simulink model "GuidanceLaw"  (R2023b)
settings: Solver=ode4  StartTime=0.0  StopTime=400  FixedStep=0.05  RelTol=1e-3
values from neighbouring files (symbols this model uses):
  APCMD_TYPE : value not decoded    [apDataDictionary.sldd]
  missionRoutePlan_struct = struct(      'validWpNum_u8', uint8(5),      'missionRoute_struct', repmat(wpDefault_struct, double(maxWpNum_u8), 1))    [initMissionRoutePlan_MC.m]
  MSSN_TYPE : value not decoded    [apDataDictionary.sldd]
  setPoint_struct = struct('lat_deg_d',double(31.200000),'lon_deg_d',double(121.500000),'alt_m_f',single(100),'yaw_deg_f',single(0))    [APTest.m]
undefined symbols (not defined in the file or in its folder): apParams
libraries: simulink x13, simulink_extras x3
(part 3 of 7)

== system GuidanceLaw/Subsystem/wpMssnHandle/GuiLaw/mcSpdGuidance/vuCmdLimit ==
  vuCmd_mps_f : Inport
  perfParams_struct : Inport  Port=2  OutDataTypeStr=Bus: perfParamBus
  curVu_mps_f : Inport  Port=3
  reset_b : Inport  Port=4
  Add : Sum  Inputs=+-
  Add1 : Sum
  Bus Selector : BusSelector  OutputSignals=maxVz_mps_f,minVz_mps_f,maxAz_mps2_f,minAz_mps2_f
  Constant : Constant  Value=apParams.dt_s_f  OutDataTypeStr=single
  Constant1 : Constant  Value=apParams.dt_s_f  OutDataTypeStr=single
  Delay : Delay  DelayLength=1
  Product : Product
  Product1 : Product
  Saturation Dynamic : simulink/Discontinuities/Saturation Dynamic  OutMin=[]  OutMax=[]  OutDataTypeStr=Inherit: Same as second input  OutDataType=fixdt(1, 16)  OutScaling=2^-10  DoSatur=off
  Saturation Dynamic2 : simulink/Discontinuities/Saturation Dynamic  OutMin=[]  OutMax=[]  OutDataTypeStr=Inherit: Same as second input  OutDataType=fixdt(1, 16)  OutScaling=2^-10  DoSatur=off
  Switch : Switch  Criteria=u2 > Threshold  SaturateOnIntegerOverflow=off  InputSameDT=off
  vuCmdLimit_mps_f : Outport
  wires:
  [vuCmdPre_mps_f] -> Switch/3
  [reset_b] -> Switch/2
  [curVu_mps_f] -> Switch/1
  Add/1 -> Saturation Dynamic/2
  Constant/1 -> Product/1
  Product/1 -> Saturation Dynamic/1
  Product1/1 -> Saturation Dynamic/3
  Constant1/1 -> Product1/2
  perfParams_struct/1 -> Bus Selector/1
  Bus Selector/1 -> [maxVu_mps_f]  "<maxVz_mps_f>"
  Bus Selector/2 -> [minVu_mps_f]  "<minVz_mps_f>"
  Bus Selector/3 -> [maxAu_mps_f]  "<maxAz_mps2_f>"
  Bus Selector/4 -> [minAu_mps_f]  "<minAz_mps2_f>"
  [maxAu_mps_f] -> Product/2
  [minAu_mps_f] -> Product1/1
  Saturation Dynamic/1 -> Add1/1
  vuCmd_mps_f/1 -> [vuCmd_mps_f]  "vuCmd_mps_f"
  [vuCmd_mps_f] -> Add/1
  Add1/1 -> Saturation Dynamic2/2
  [maxVu_mps_f] -> Saturation Dynamic2/1
  [minVu_mps_f] -> Saturation Dynamic2/3
  Saturation Dynamic2/1 -> Delay/1, vuCmdLimit_mps_f/1
  Delay/1 -> [vuCmdPre_mps_f]
  curVu_mps_f/1 -> [curVu_mps_f]
  reset_b/1 -> [reset_b]  "reset_b"
  Switch/1 -> Add1/2, Add/2

== system GuidanceLaw/Subsystem/wpMssnHandle/GuiLaw/mcSpdGuidance/vxCmdLimit ==
  vxCmd_mps_f : Inport
  perfParams_struct : Inport  Port=2  OutDataTypeStr=Bus: perfParamBus
  curVx_mps_f : Inport  Port=3
  reset_b : Inport  Port=4
  Add : Sum  Inputs=+-
  Add1 : Sum
  Bus Selector : BusSelector  OutputSignals=maxVx_mps_f,minVx_mps_f,maxAx_mps2_f,minAx_mps2_f
  Constant : Constant  Value=apParams.dt_s_f  OutDataTypeStr=single
  Constant1 : Constant  Value=apParams.dt_s_f  OutDataTypeStr=single
  Delay : Delay  DelayLength=1
  Product : Product
  Product1 : Product
  Saturation Dynamic : simulink/Discontinuities/Saturation Dynamic  OutMin=[]  OutMax=[]  OutDataTypeStr=Inherit: Same as second input  OutDataType=fixdt(1, 16)  OutScaling=2^-10  DoSatur=off
  Saturation Dynamic2 : simulink/Discontinuities/Saturation Dynamic  OutMin=[]  OutMax=[]  OutDataTypeStr=Inherit: Same as second input  OutDataType=fixdt(1, 16)  OutScaling=2^-10  DoSatur=off
  Switch : Switch  Criteria=u2 > Threshold  SaturateOnIntegerOverflow=off  InputSameDT=off
  vxCmdLimit_mps_f : Outport
  wires:
  [vxCmdPre_mps_f] -> Switch/3
  [reset_b] -> Switch/2
  [curVx_mps_f] -> Switch/1
  Add/1 -> Saturation Dynamic/2
  Constant/1 -> Product/1
  Product/1 -> Saturation Dynamic/1
  Product1/1 -> Saturation Dynamic/3
  Constant1/1 -> Product1/2
  perfParams_struct/1 -> Bus Selector/1
  Bus Selector/1 -> [maxVx_mps_f]  "<maxVx_mps_f>"
  Bus Selector/2 -> [minVx_mps_f]  "<minVx_mps_f>"
  Bus Selector/3 -> [maxAx_mps_f]  "<maxAx_mps2_f>"
  Bus Selector/4 -> [minAx_mps_f]  "<minAx_mps2_f>"
  [maxAx_mps_f] -> Product/2
  [minAx_mps_f] -> Product1/1
  Saturation Dynamic/1 -> Add1/1
  vxCmd_mps_f/1 -> [vxCmd_mps_f]
  [vxCmd_mps_f] -> Add/1
  Add1/1 -> Saturation Dynamic2/2
  [maxVx_mps_f] -> Saturation Dynamic2/1
  [minVx_mps_f] -> Saturation Dynamic2/3
  Saturation Dynamic2/1 -> Delay/1, vxCmdLimit_mps_f/1
  Delay/1 -> [vxCmdPre_mps_f]
  curVx_mps_f/1 -> [curVx_mps_f]
  reset_b/1 -> [reset_b]
  Switch/1 -> Add1/2, Add/2

== system GuidanceLaw/Subsystem/wpMssnHandle/GuiLaw/mcSpdGuidance/vyCmdLimit ==
  vyCmd_mps_f : Inport
  perfParams_struct : Inport  Port=2  OutDataTypeStr=Bus: perfParamBus
  curVy_mps_f : Inport  Port=3
  reset_b : Inport  Port=4
  Add : Sum  Inputs=+-
  Add1 : Sum
  Bus Selector : BusSelector  OutputSignals=maxVy_mps_f,minVy_mps_f,maxAy_mps2_f,minAy_mps2_f
  Constant : Constant  Value=apParams.dt_s_f  OutDataTypeStr=single
  Constant1 : Constant  Value=apParams.dt_s_f  OutDataTypeStr=single
  Delay : Delay  DelayLength=1
  Product : Product
  Product1 : Product
  Saturation Dynamic : simulink/Discontinuities/Saturation Dynamic  OutMin=[]  OutMax=[]  OutDataTypeStr=Inherit: Same as second input  OutDataType=fixdt(1, 16)  OutScaling=2^-10  DoSatur=off
  Saturation Dynamic2 : simulink/Discontinuities/Saturation Dynamic  OutMin=[]  OutMax=[]  OutDataTypeStr=Inherit: Same as second input  OutDataType=fixdt(1, 16)  OutScaling=2^-10  DoSatur=off
  Switch : Switch  Criteria=u2 > Threshold  SaturateOnIntegerOverflow=off  InputSameDT=off
  vyCmdLimit_mps_f : Outport
  wires:
  [vyCmdPre_mps_f] -> Switch/3
  [reset_b] -> Switch/2
  [curVy_mps_f] -> Switch/1
  Add/1 -> Saturation Dynamic/2
  Constant/1 -> Product/1
  Product/1 -> Saturation Dynamic/1
  Product1/1 -> Saturation Dynamic/3
  Constant1/1 -> Product1/2
  perfParams_struct/1 -> Bus Selector/1
  Bus Selector/1 -> [maxVy_mps_f]  "<maxVy_mps_f>"
  Bus Selector/2 -> [minVy_mps_f]  "<minVy_mps_f>"
  Bus Selector/3 -> [maxAy_mps_f]  "<maxAy_mps2_f>"
  Bus Selector/4 -> [minAy_mps_f]  "<minAy_mps2_f>"
  [maxAy_mps_f] -> Product/2
  [minAy_mps_f] -> Product1/1
  Saturation Dynamic/1 -> Add1/1
  vyCmd_mps_f/1 -> [vyCmd_mps_f]
  [vyCmd_mps_f] -> Add/1
  Add1/1 -> Saturation Dynamic2/2
  [maxVy_mps_f] -> Saturation Dynamic2/1
  [minVy_mps_f] -> Saturation Dynamic2/3
  Saturation Dynamic2/1 -> Delay/1, vyCmdLimit_mps_f/1
  Delay/1 -> [vyCmdPre_mps_f]
  curVy_mps_f/1 -> [curVy_mps_f]
  reset_b/1 -> [reset_b]
  Switch/1 -> Add/2, Add1/2

== system GuidanceLaw/Subsystem/wpMssnHandle/GuiLaw/yawGuidance/yawCmdLimit ==
  yawCmd_deg_f : Inport
  perfParams_struct : Inport  Port=2  OutDataTypeStr=Bus: perfParamBus
  curYaw_deg_f : Inport  Port=3
  reset_b : Inport  Port=4
  Add : Sum  Inputs=+-
  Add1 : Sum
  Bus Selector : BusSelector  OutputSignals=maxYawAngleRate_dps_f,minYawAngleRate_dps_f
  Constant : Constant  Value=apParams.dt_s_f  OutDataTypeStr=single
  Constant1 : Constant  Value=apParams.dt_s_f  OutDataTypeStr=single
  Delay : Delay  DelayLength=1
  Product : Product
  Product1 : Product
  Saturation Dynamic : simulink/Discontinuities/Saturation Dynamic  OutMin=[]  OutMax=[]  OutDataTypeStr=Inherit: Same as second input  OutDataType=fixdt(1, 16)  OutScaling=2^-10  DoSatur=off
  Switch : Switch  Criteria=u2 > Threshold  SaturateOnIntegerOverflow=off  InputSameDT=off
  cldWrap180 : MATLAB Function  TreatAsAtomicUnit=on
  cldWrap1801 : MATLAB Function  TreatAsAtomicUnit=on
  yawCmdLimit_deg_f : Outport
  wires:
  [yawCmdPre_mps_f] -> Switch/3
  [reset_b] -> Switch/2
  [curYaw_deg_f] -> Switch/1
  Constant/1 -> Product/1
  Product/1 -> Saturation Dynamic/1
  Product1/1 -> Saturation Dynamic/3
  Constant1/1 -> Product1/2
  perfParams_struct/1 -> Bus Selector/1
  Bus Selector/1 -> [maxYawRate_dps_f]  "<maxYawAngleRate_dps_f>"
  Bus Selector/2 -> [minYawRate_dps_f]  "<minYawAngleRate_dps_f>"
  [maxYawRate_dps_f] -> Product/2
  [minYawRate_dps_f] -> Product1/1
  Saturation Dynamic/1 -> Add1/1
  yawCmd_deg_f/1 -> [yawCmd_deg_f]
  [yawCmd_deg_f] -> Add/1
  cldWrap1801/1(y) -> Delay/1, yawCmdLimit_deg_f/1
  Delay/1 -> [yawCmdPre_mps_f]
  curYaw_deg_f/1 -> [curYaw_deg_f]
  reset_b/1 -> [reset_b]
  Switch/1 -> Add1/2, Add/2
  cldWrap180/1(y) -> Saturation Dynamic/2
  Add/1 -> cldWrap180/1(u)
  Add1/1 -> cldWrap1801/1(u)

== system GuidanceLaw/Subsystem/wpMssnHandle/WaypointArrivalState/hoverYawJudge/YawAlignJudge ==
  note: 仅当 isHoverPosReach_b=true 时执行。
      | 禁用时输出复位为 false，重新使能时内部状态复位。
  curPosNEU_m_f : Inport
  curYaw_deg_f : Inport  Port=2
  reset_b : Inport  Port=3
  nextWp_struct : Inport  Port=4
  curWp_struct : Inport  Port=5
  Enable : EnablePort  StatesWhenEnabling=reset
  Bus Selector : BusSelector  OutputSignals=yawType_u8,yaw_deg_f,posN_m_f,posE_m_f
  Bus Selector1 : BusSelector  OutputSignals=posN_m_f,posE_m_f
  Constant1 : Constant  Value=apParams.hoverYawJudge.holdTimeCond_s_f  OutDataTypeStr=single
  Constant2 : Constant  Value=apParams.hoverYawJudge.minYawDirDist_m_f  OutDataTypeStr=single
  Constant21 : Constant  Value=apParams.dt_s_f  OutDataTypeStr=single
  Constant9 : Constant  Value=apParams.hoverYawJudge.yawTolerance_deg_f  OutDataTypeStr=single
  Selector : Selector  InputPortWidth=3  IndexOptions=Index vector (dialog)  Indices=[1 2]  OutputSizes=1
  Terminator : Terminator
  Vector Concatenate : Concatenate
  Vector Concatenate1 : Concatenate
  YawJudgeAlgorithmBlock : MATLAB Function  TreatAsAtomicUnit=on
  hoverYawJudge_b : Outport  OutDataTypeStr=boolean  OutputWhenDisabled=reset  InitialOutput=false
  wires:
  YawJudgeAlgorithmBlock/1(hoverYawJudge_b) -> hoverYawJudge_b/1
  YawJudgeAlgorithmBlock/2(yawCmd_deg_f) -> Terminator/1
  curYaw_deg_f/1 -> YawJudgeAlgorithmBlock/3(curYaw_deg_f)
  Constant21/1 -> YawJudgeAlgorithmBlock/7(dt_s_f)
  Constant9/1 -> YawJudgeAlgorithmBlock/8(yawErrAccept_deg_f)
  Constant1/1 -> YawJudgeAlgorithmBlock/9(holdTimeYaw_s_f)
  Constant2/1 -> YawJudgeAlgorithmBlock/10(minYawDirDist_m_f)
  reset_b/1 -> YawJudgeAlgorithmBlock/6(reset_b)
  nextWp_struct/1 -> Bus Selector/1
  Bus Selector/1 -> [nextWpYawType_u8]  "<yawType_u8>"
  [nextWpYawType_u8] -> YawJudgeAlgorithmBlock/4(nextWpYawType_u8)
  Bus Selector/2 -> [nextWpYaw_deg_f]  "<yaw_deg_f>"
  [nextWpYaw_deg_f] -> YawJudgeAlgorithmBlock/5(nextWpYaw_deg_f)
  Bus Selector/3 -> Vector Concatenate/1  "<posN_m_f>"
  Bus Selector/4 -> Vector Concatenate/2  "<posE_m_f>"
  Vector Concatenate/1 -> [nextWpNE_m_f]
  [nextWpNE_m_f] -> YawJudgeAlgorithmBlock/2(nextWpNE_m_f)
  curWp_struct/1 -> Bus Selector1/1
  Bus Selector1/1 -> Vector Concatenate1/1  "<posN_m_f>"
  Bus Selector1/2 -> Vector Concatenate1/2  "<posE_m_f>"
  Vector Concatenate1/1 -> [curWpNE_m_f]
  [curWpNE_m_f] -> YawJudgeAlgorithmBlock/11(curWpNE_m_f)
  curPosNEU_m_f/1 -> [curPosNEU_m_f]
  Selector/1 -> YawJudgeAlgorithmBlock/1(curPosNE_m_f)
  [curPosNEU_m_f] -> Selector/1

== matlab function GuidanceLaw/Subsystem/wpMssnHandle/GuiLaw/L1CirleGuidance/L1CirleGuidance ==
  data: kdCir_f input; rollCmd_deg_f output; ktCir_f input; curVelNE_mps_f input; curPosNE_mps_f input; velXY_min input; G_mps2_f input; curPitch_deg_f input; curGpPosN_m_f input; curWpPosE_m_f input; curWpRadius_m_f input; circle_radius_min input; curYaw_deg_f input
function rollCmd_deg_f = l1CircleGuidance(kdCir_f, ktCir_f, curVelNE_mps_f, curPosNE_mps_f, velXY_min, G_mps2_f, curPitch_deg_f, curGpPosN_m_f, ...
    curWpPosE_m_f, curWpRadius_m_f, circle_radius_min, curYaw_deg_f)
%L1圆弧导引算法
%
% 优化内容：
% 1. 全部内部计算统一为single，便于Simulink代码生成。
% 2. 增加周期、阻尼、重力、半径、速度和距离的有效性保护。
% 3. 避免飞机位于圆心时出现除零。
% 4. 使用显式二维运算替代norm/dot/辅助函数，计算量和类型更可控。
% 5. 低速时使用当前偏航方向构造等效速度。
% 6. 启用30 deg滚转角限幅，可按机型修改ROLL_LIMIT_DEG。
% 7. 圆周向心加速度使用真实有效半径，不再隐式限制为至少1 m。
%
% 输入：
%   curVelNE_mps_f = [v_N, v_E]，m/s，1×2
%   curPosNE_mps_f = [p_N, p_E]，m，1×2
%   curWpRadius_m_f > 0：顺时针；< 0：逆时针
%
%#codegen

%--------------------------- 常量定义 ------------------------------------
ZERO = single(0);
ONE  = single(1);
TWO  = single(2);
FOUR = single(4);

PI_S      = single(pi);
DEG2RAD_S = PI_S / single(180);
RAD2DEG_S = single(180) / PI_S;

EPS_PARAM = single(1.0e-6);
EPS_DIST  = single(1.0e-3);

% 默认安全输出
rollCmd_deg_f = ZERO;

%--------------------------- 输入类型统一 --------------------------------
Kd       = single(kdCir_f);
T_period = single(ktCir_f);
g        = single(G_mps2_f);

vN = single(curVelNE_mps_f(1));
vE = single(curVelNE_mps_f(2));

posN = single(curPosNE_mps_f(1));
posE = single(curPosNE_mps_f(2));

centerN = single(curGpPosN_m_f);
centerE = single(curWpPosE_m_f);

radius_cmd = single(curWpRadius_m_f);
radius_min = abs(single(circle_radius_min));
v_min      = max(single(velXY_min), ZERO);

yaw_rad   = single(curYaw_deg_f)   * DEG2RAD_S;
pitch_rad = single(curPitch_deg_f) * DEG2RAD_S;

%--------------------------- 参数有效性检查 ------------------------------
if Kd <= EPS_PARAM || T_period <= EPS_PARAM || g <= EPS_PARAM
    return;
end

% 带符号半径决定盘旋方向
if radius_cmd > EPS_PARAM
    loiter_direction = ONE;       % 顺时针
elseif radius_cmd < -EPS_PARAM
    loiter_direction = -ONE;      % 逆时针
else
    % 半径无方向信息，禁止产生不确定的盘旋指令
    return;
end

radius = max(abs(radius_cmd), max(radius_min, EPS_DIST));

%--------------------------- 地速处理 ------------------------------------
groundspeed_sq = vN * vN + vE * vE;
groundspeed = sqrt(max(groundspeed_sq, ZERO));

% 低速时，用当前偏航方向构造最小等效地速
if groundspeed < v_min
    groundspeed = v_min;
    vN = groundspeed * cos(yaw_rad);
    vE = groundspeed * sin(yaw_rad);
end

% 速度仍接近0时无法形成有效L1导引
if groundspeed <= EPS_PARAM
    return;
end

%--------------------------- L1参数计算 ----------------------------------
omega = TWO * PI_S / T_period;
K_c   = omega * omega;
K_v   = TWO * Kd * omega;
k_r   = Kd * T_period / PI_S;
K_L1  = FOUR * Kd * Kd;

L1 = k_r * groundspeed;
if L1 <= EPS_PARAM
    return;
end

%--------------------------- 圆心方向计算 --------------------------------
% 位置指向圆心：P -> C
dN = centerN - posN;
dE = centerE - posE;

distance_sq = dN * dN + dE * dE;
distance_to_center = sqrt(max(distance_sq, ZERO));

if distance_to_center > EPS_DIST
    inv_distance = ONE / distance_to_center;
    unitN = dN * inv_distance;
    unitE = dE * inv_distance;
else
    % 飞机恰好位于圆心，P->C方向不确定。
    % 构造一个与当前速度垂直、且与目标旋转方向一致的单位方向，
    % 使算法能够主动建立盘旋，而不是产生NaN。
    inv_speed = ONE / groundspeed;
    unitN = -loiter_direction * vE * inv_speed;
    unitE =  loiter_direction * vN * inv_speed;
    distance_to_center = ZERO;
end

% 速度在P->C方向上的横向和纵向分量
xtrackVelCap = vN * unitE - vE * unitN;
ltrackVelCap = vN * unitN + vE * unitE;

%--------------------------- 圆心捕获L1导引 ------------------------------
eta = atan2(xtrackVelCap, ltrackVelCap);
eta = min(max(eta, -PI_S / TWO), PI_S / TWO);

latAccDemLine = K_L1 * groundspeed * groundspeed / L1 * sin(eta);

%--------------------------- 圆航线跟踪 ----------------------------------
% 径向误差：圆外为正，圆内为负
xtrackErrCirc = distance_to_center - radius;

% 径向速度：向圆外运动为正，向圆心运动为负
xtrackVelCirc = -ltrackVelCap;

% 径向PD修正项
latAccDemCircPD = K_c * xtrackErrCirc + K_v * xtrackVelCirc;

% 与目标盘旋方向一致的切向速度
velTangent = loiter_direction * xtrackVelCap;

% 当前速度方向与目标盘旋方向相反时，
% 禁止PD项继续诱导飞机向反方向旋转
if ltrackVelCap < ZERO && velTangent < ZERO
    latAccDemCircPD = max(ZERO, latAccDemCircPD);
end

% 圆周跟踪指令 = 径向PD修正 + 向心加速度前馈
latAccDemCirc = loiter_direction * (latAccDemCircPD + velTangent * velTangent / radius);

%--------------------------- 捕获/跟踪切换 -------------------------------
% 飞机位于圆外时，若圆心捕获指令更温和，则采用捕获指令；
% 否则直接采用圆航线跟踪指令。
if xtrackErrCirc > ZERO && loiter_direction * latAccDemLine < loiter_direction * latAccDemCirc
    lateral_accel = latAccDemLine;
else
    lateral_accel = latAccDemCirc;
end

%--------------------------- 滚转角反算 ----------------------------------
roll_rad = atan(cos(pitch_rad) * lateral_accel / g);
rollCmd_deg_f = single(roll_rad * RAD2DEG_S);

end

== matlab function GuidanceLaw/Subsystem/wpMssnHandle/GuiLaw/L1LineGuidance/L1LineGuidance ==
  data: kdLine_f input; rollCmd_deg_f output; ktLine_f input; curVelNE_mps_f input; curPosNE_m_f input; velXY_min input; G_mps2_f input; curPitch_deg_f input; curGpPosN_m_f input; curGpPosE_m_f input; preGpPosN_m_f input; preGpPosE_m_f input; mssnType_u8 input; curYaw_deg_f input
function rollCmd_deg_f = l1LineGuidance(kdLine_f, ktLine_f, curVelNE_mps_f, curPosNE_m_f, velXY_min, G_mps2_f, curPitch_deg_f, curGpPosN_m_f, curGpPosE_m_f, preGpPosN_m_f, ...
    preGpPosE_m_f, mssnType_u8, curYaw_deg_f)
%#codegen
%
% 坐标约定：
%   水平面N-E坐标
%   curVelNE_mps_f = [VN, VE]
%   curPosNE_m_f   = [PN, PE]
%
% 输出：
%   rollCmd_deg_f，单位deg

%% 常量
PI_F       = single(3.14159265358979323846);
DEG2RAD_F  = single(0.01745329251994329577);
RAD2DEG_F  = single(57.2957795130823208768);

EPS_DIST   = single(1.0e-6);
EPS_SPEED  = single(1.0e-3);
EPS_G      = single(1.0e-3);

L1_MIN     = single(0.1);
SIN_45     = single(0.7071067811865476);
ETA_MAX    = single(0.5) * PI_F;
ANGLE_100  = single(100.0) * DEG2RAD_F;

rollCmd_deg_f = single(0.0);

%% 参数有效性保护
if (kdLine_f <= single(0.0)) || (ktLine_f <= single(0.0)) || (G_mps2_f <= EPS_G)
    return;
end

%% 读取当前位置、速度和航点
vN = curVelNE_mps_f(1);
vE = curVelNE_mps_f(2);

pN = curPosNE_m_f(1);
pE = curPosNE_m_f(2);

% 航段起点A
aN = preGpPosN_m_f;
aE = preGpPosE_m_f;

% 航段终点B
bN = curGpPosN_m_f;
bE = curGpPosE_m_f;

%% 计算当前地速
groundSpeedSq = vN * vN + vE * vE;
groundSpeed   = sqrt(groundSpeedSq);

% 最小地速限制
speedFloor = max(velXY_min, EPS_SPEED);

if groundSpeed < speedFloor
    groundSpeed = speedFloor;

    % 当前速度过小时，使用当前偏航角构造虚拟速度
    yaw_rad = curYaw_deg_f * DEG2RAD_F;

    vN = groundSpeed * cos(yaw_rad);
    vE = groundSpeed * sin(yaw_rad);
end

%% L1参数
k_r  = kdLine_f * ktLine_f / PI_F;
k_L1 = single(4.0) * kdLine_f * kdLine_f;

% L1距离增加下限保护
L1 = max(k_r * groundSpeed, L1_MIN);

%% 计算航段方向A->B
abN = bN - aN;
abE = bE - aE;

abLength = sqrt(abN * abN + abE * abE);

% 如果航段A、B重合，则退化为当前位置直接指向B
if abLength < EPS_DIST
    abN = bN - pN;
    abE = bE - pE;

    abLength = sqrt(abN * abN + abE * abE);

    % 当前位置也在B点，直接输出零
    if abLength < EPS_DIST
        return;
    end
end

% 航段方向单位向量
dirAbN = abN / abLength;
dirAbE = abE / abLength;

%% P指向A
paN = aN - pN;
paE = aE - pE;

distancePtoA = sqrt(paN * paN + paE * paE);

% A指向P
apN = -paN;
apE = -paE;

% 当前点在航段方向上的投影
trackDist = apN * dirAbN + apE * dirAbE;

%% P指向B
pbN = bN - pN;
pbE = bE - pE;

distancePtoB = sqrt(pbN * pbN + pbE * pbE);

%% 前倾飞行状态判断
% 如果项目中没有MSSN_TYPE枚举，需要将右侧替换为实际枚举值。
isForwardTilt = (mssnType_u8 == MSSN_TYPE.AUTO_FORWARD_TILT);

%% 判断是否位于A点后方
beforeARatio = trackDist / max(distancePtoA, single(1.0));

useDirectToA = (~isForwardTilt) && (distancePtoA > L1) && (beforeARatio < -SIN_45);

%% 判断是否位于B点外侧区域
useDirectToB = false;

if distancePtoB > EPS_DIST
    % B指向P的单位向量
    bpN = -pbN / distancePtoB;
    bpE = -pbE / distancePtoB;

    % BP到AB的有符号夹角
    crossBpAb = cross2(bpN, bpE, dirAbN, dirAbE);
    dotBpAb   = bpN * dirAbN + bpE * dirAbE;

    bpToAbBearing = atan2(crossBpAb, dotBpAb);

    useDirectToB = (~isForwardTilt) && (abs(bpToAbBearing) < ANGLE_100);
end

%% 计算导引角eta
if useDirectToA
    % 飞向A点
    targetN = paN / distancePtoA;
    targetE = paE / distancePtoA;

    eta = signedAngle(vN, vE, targetN, targetE);

elseif useDirectToB
    % 飞向B点
    targetN = pbN / distancePtoB;
    targetE = pbE / distancePtoB;

    eta = signedAngle(vN, vE, targetN, targetE);

else
    % 当前速度方向与航段方向的夹角
    eta2 = signedAngle(vN, vE, dirAbN, dirAbE);

    % 有符号横向航迹误差
    %
    % error_d = cross(A->P, A->B单位向量)
    error_d = cross2(apN, apE, dirAbN, dirAbE);

    % 横向误差转化为捕获角
    sineEta1 = error_d / L1;

    % 捕获角限制为±45°
    sineEta1 = constrain_scalar(sineEta1, -SIN_45, SIN_45);

    eta1 = asin(sineEta1);

    eta = eta1 + eta2;
end

%% 限制总导引角
eta = constrain_scalar(eta, -ETA_MAX, ETA_MAX);

%% 计算侧向加速度
lateralAccel = k_L1 * groundSpeed * groundSpeed / L1 * sin(eta);

%% 侧向加速度转换为滚转角
pitch_rad = curPitch_deg_f * DEG2RAD_F;

roll_rad = atan2(cos(pitch_rad) * lateralAccel, G_mps2_f);

rollCmd_deg_f = single(roll_rad * RAD2DEG_F);

end


function c = cross2(aN, aE, bN, bE)
% 二维叉乘
c = aN * bE - aE * bN;
end


function angle = signedAngle(aN, aE, bN, bE)
% 从向量a旋转到向量b的有符号夹角
crossValue = aN * bE - aE * bN;
dotValue   = aN * bN + aE * bE;

angle = atan2(crossValue, dotValue);
end


% function y = clampLimit(x, lowerLimit, upperLimit)
% % 上下限约束
% y = min(max(x, lowerLimit), upperLimit);
% end

== matlab function GuidanceLaw/Subsystem/wpMssnHandle/GuiLaw/mcSpdGuidance/mcTrajectoryGeneratorNEU/TrajectoryGeneratorNEU ==
  data: trajPosNEU_m_f output; curPosNEU_m_f input; curVelNEU_mps_f input; curAccNEU_mps2_f input; preWpNEU_m_f input; curWpNEU_m_f input; nextWpNEU_m_f input; velSpNEU_mps_f input; posVelValid_vec input; isHoverWp_b input; forceStop_b input; segSwitch_b input; newOriOldNEU_m_f input; dt_s_f input; reset_b input; paramNE_f input; trajVelNEU_mps_f output; trajAccNEU_mps2_f output; trajJerkNEU_mps3_f output; paramU_f input
function [trajPosNEU_m_f, trajVelNEU_mps_f, trajAccNEU_mps2_f, trajJerkNEU_mps3_f] = trajGeneratorNEU(curPosNEU_m_f, curVelNEU_mps_f, curAccNEU_mps2_f, preWpNEU_m_f, curWpNEU_m_f, nextWpNEU_m_f, ...
    velSpNEU_mps_f, posVelValid_vec, isHoverWp_b, forceStop_b, segSwitch_b, newOriOldNEU_m_f, dt_s_f, reset_b, paramNE_f, paramU_f)
%#codegen
%
% 功能：
% 生成NEU三轴jerk受限平滑轨迹，并进行N/E/U三轴S曲线时间同步。
%
% velSpNEU_mps_f：
% 1. 对应位置无效时，为纯速度目标；
% 2. 对应位置有效时，为位置导引速度上的速度前馈。
%
% posVelValid_vec：[posNEValid; velNEValid; posUValid; velUValid]
%
% paramNE_f：
% 1 最大水平jerk，[m/s^3]
% 2 最大水平加速度，[m/s^2]
% 3 最大水平速度，[m/s]
% 4 水平巡航速度，[m/s]
% 5 最大允许水平轨迹误差，[m]
% 6 水平航点接受半径，[m]
% 7 最小前视距离，[m]
% 8 转弯判断最小轨迹速度，[m/s]
% 9 转弯判断方向余弦阈值
% 10 前倾转换阶段旋翼水平速度，[m/s]
% 11 旋翼直线最小提前判定距离，[m]
% 12 旋翼直线最大提前判定距离，[m]
% 13 旋翼直线相邻航段长度限制比例，建议<=0.49
%
% paramU_f：
% 1 最大垂向jerk，[m/s^3]
% 2 爬升轨迹使用的最大垂向加速度幅值，[m/s^2]
% 3 下降轨迹使用的最大垂向加速度幅值，[m/s^2]
% 4 最大爬升速度，[m/s]
% 5 最大下降速度幅值，[m/s]
% 6 最大允许垂向轨迹误差，[m]
% 7 垂向航点接受半径，[m]
%
% 垂向非对称约束：
% 1. 根据未平滑垂向速度目标rawVelSpNEU_mps_f(3)的方向，选择一整套
%    垂向速度和加速度幅值约束；
% 2. 选定后，单轴S曲线规划器内部仍使用对称的+/-maxAcceleration约束；
% 3. rawVelSpU为0时保持上一套约束，避免停车附近反复切换。

%% 常量

smallValue_f = single(1.0e-6);
floatEpsilon_f = single(1.1920929e-7);
clampAccuracy_mps_f = single(0.5);

%% 最小持久状态
% 轨迹生成器每个周期都会根据当前状态重新规划S曲线，并在同一周期推进dt。
persistent trajAccStateNEU_mps2_f trajVelStateNEU_mps_f trajPosStateNEU_m_f
persistent selectedUConstraintModeState_i8
persistent preMaxSpeedNEState_mps_f
persistent turnJudgeDistState_m_f turnPassSpeedState_mps_f
persistent initialized_b

if isempty(initialized_b)
    initialized_b = false;

    trajAccStateNEU_mps2_f = single(zeros(3,1));
    trajVelStateNEU_mps_f = single(zeros(3,1));
    trajPosStateNEU_m_f = single(zeros(3,1));
    selectedUConstraintModeState_i8 = int8(0);
    preMaxSpeedNEState_mps_f = single(0.0);
    turnJudgeDistState_m_f = single(0.0);
    turnPassSpeedState_mps_f = single(0.0);
end

%% 参数读取
maxJerkNE_mps3_f = max(paramNE_f(1), smallValue_f);
maxAccNE_mps2_f = max(paramNE_f(2), smallValue_f);
maxVelNE_mps_f = max(paramNE_f(3), smallValue_f);
maxRouteSpeedNE_mps_f = constrain_scalar(paramNE_f(4), single(0.0), maxVelNE_mps_f);
maxTrajErrorNE_m_f = max(paramNE_f(5), smallValue_f);
horizonAptRadius_m_f = max(paramNE_f(6), smallValue_f);
minLookaheadDist_m_f = max(paramNE_f(7), horizonAptRadius_m_f);
turnMinSpeed_mps_f = max(paramNE_f(8), single(0.0));
turnCosThreshold_f = constrain_scalar(paramNE_f(9), single(-1.0), single(1.0));
fwdFixedSpd_mps_f = max(paramNE_f(10), smallValue_f);
minJudgeDistNE_m_f = max(paramNE_f(11), single(0.0));
maxJudgeDistNE_m_f = max(paramNE_f(12), minJudgeDistNE_m_f);
segmentLimitRatioNE_f = min(max(paramNE_f(13), single(0.0)), single(0.49));

maxJerkU_mps3_f = max(paramU_f(1), smallValue_f);
maxAccUp_mps2_f = max(paramU_f(2), smallValue_f);
maxAccDown_mps2_f = max(paramU_f(3), smallValue_f);
maxVelUp_mps_f = max(paramU_f(4), smallValue_f);
maxVelDown_mps_f = max(paramU_f(5), smallValue_f);
maxTrajErrorU_m_f = max(paramU_f(6), smallValue_f);
verticalAcceptanceRadius_m_f = max(paramU_f(7), smallValue_f);

axisMaxJerkNEU_mps3_f = single([maxJerkNE_mps3_f; maxJerkNE_mps3_f; maxJerkU_mps3_f]);

dtEff_s_f = max(dt_s_f, single(0.0));

%% 输入有效性
posNEValid_b = logical(posVelValid_vec(1));
velNEValid_b = logical(posVelValid_vec(2));
posUValid_b = logical(posVelValid_vec(3));
velUValid_b = logical(posVelValid_vec(4));

%% 初始化、复位或航段坐标系切换
if reset_b || ~initialized_b
    trajAccStateNEU_mps2_f = curAccNEU_mps2_f;
    trajVelStateNEU_mps_f = curVelNEU_mps_f;
    trajPosStateNEU_m_f = curPosNEU_m_f;

    trajAccStateNEU_mps2_f(1) = constrain_scalar(curAccNEU_mps2_f(1), -maxAccNE_mps2_f, maxAccNE_mps2_f);
    trajAccStateNEU_mps2_f(2) = constrain_scalar(curAccNEU_mps2_f(2), -maxAccNE_mps2_f, maxAccNE_mps2_f);
    trajAccStateNEU_mps2_f(3) = constrain_scalar(curAccNEU_mps2_f(3), -maxAccDown_mps2_f, maxAccUp_mps2_f);

    trajVelStateNEU_mps_f(1) = constrain_scalar(curVelNEU_mps_f(1), -maxVelNE_mps_f, maxVelNE_mps_f);
    trajVelStateNEU_mps_f(2) = constrain_scalar(curVelNEU_mps_f(2), -maxVelNE_mps_f, maxVelNE_mps_f);
    trajVelStateNEU_mps_f(3) = constrain_scalar(curVelNEU_mps_f(3), -maxVelDown_mps_f, maxVelUp_mps_f);

    % 1表示爬升约束，-1表示下降约束，0表示尚未选择方向并采用保守值。
    if curVelNEU_mps_f(3) > smallValue_f
        selectedUConstraintModeState_i8 = int8(1);
    elseif curVelNEU_mps_f(3) < -smallValue_f
        selectedUConstraintModeState_i8 = int8(-1);
    else
        selectedUConstraintModeState_i8 = int8(0);
    end

    preMaxSpeedNEState_mps_f = single(0.0);

    [turnJudgeDistState_m_f, turnPassSpeedState_mps_f] = computeMcTurnConstraint(preWpNEU_m_f(1:2), curWpNEU_m_f(1:2), nextWpNEU_m_f(1:2), maxRouteSpeedNE_mps_f, maxAccNE_mps2_f, ...
        minJudgeDistNE_m_f, maxJudgeDistNE_m_f, segmentLimitRatioNE_f, smallValue_f);
    initialized_b = true;

elseif segSwitch_b
    % 各航段坐标轴方向不变，仅平移原点。
    % 速度和加速度状态保持连续，只更新位置原点。
    trajPosStateNEU_m_f = trajPosStateNEU_m_f - newOriOldNEU_m_f;

    % 航段切换后，基于新的pre-cur-next冻结下一航点转弯约束。
    [turnJudgeDistState_m_f, turnPassSpeedState_mps_f] = computeMcTurnConstraint(preWpNEU_m_f(1:2), curWpNEU_m_f(1:2), nextWpNEU_m_f(1:2), maxRouteSpeedNE_mps_f, maxAccNE_mps2_f, ...
        minJudgeDistNE_m_f, maxJudgeDistNE_m_f, segmentLimitRatioNE_f, smallValue_f);
else
    % 不处理
end

%% 按有效性组合生成原始速度目标

% 先装载速度输入。位置有效时，它是位置速度的前馈；位置无效时，
% 它就是直接送给S曲线平滑器的纯速度目标。无效速度分量保持为0。
rawVelSpNEU_mps_f = single(zeros(3,1));

if velNEValid_b
    rawVelSpNEU_mps_f(1:2) = velSpNEU_mps_f(1:2);
end

if velUValid_b
    rawVelSpNEU_mps_f(3) = velSpNEU_mps_f(3);
end

if forceStop_b
    % 强制停车优先级最高，忽略位置目标和速度前馈。
    rawVelSpNEU_mps_f = single(zeros(3,1));

elseif posNEValid_b && posUValid_b
    %% NE和U位置同时有效：生成三维位置速度目标
    waypointsNEU_m_f = [preWpNEU_m_f, curWpNEU_m_f, nextWpNEU_m_f];

    [crossingPointNEU_m_f, targetSpeedNE_mps_f, preMaxSpeedNEState_mps_f] = get_xy_guidance_constraints_handle(trajPosStateNEU_m_f, trajVelStateNEU_mps_f, waypointsNEU_m_f, ...
        isHoverWp_b, maxRouteSpeedNE_mps_f, maxJerkNE_mps3_f, maxAccNE_mps2_f, horizonAptRadius_m_f, minLookaheadDist_m_f, turnMinSpeed_mps_f, ...
        turnCosThreshold_f, turnJudgeDistState_m_f, turnPassSpeedState_mps_f, preMaxSpeedNEState_mps_f, smallValue_f);

    if isHoverWp_b
        nextWpForUSpeed_m_f = curWpNEU_m_f(3);
    else
        nextWpForUSpeed_m_f = nextWpNEU_m_f(3);
    end

    maxAllowedSpeedU_mps_f = get_max_z_speed_handle(trajPosStateNEU_m_f(3), curWpNEU_m_f(3), nextWpForUSpeed_m_f, maxJerkU_mps3_f, maxAccUp_mps2_f, maxAccDown_mps2_f, ...
        maxVelUp_mps_f, maxVelDown_mps_f, verticalAcceptanceRadius_m_f, smallValue_f);

    posToCrossingNEU_m_f = crossingPointNEU_m_f - trajPosStateNEU_m_f;
    directionToCrossingNEU_f = unit_or_zero(posToCrossingNEU_m_f, smallValue_f);
    combinedSpeed_mps_f = sqrt(targetSpeedNE_mps_f * targetSpeedNE_mps_f + maxAllowedSpeedU_mps_f * maxAllowedSpeedU_mps_f);
    posVelSpNEU_mps_f = directionToCrossingNEU_f * combinedSpeed_mps_f;

    % 先限制水平模长，再限制垂向模长。
    % clampAccuracy_mps_f = 0.5是小速度区间判定精度accuracy，不是另一方向的固定缩放系数。
    posVelSpNEU_mps_f = clamp_to_xy_norm(posVelSpNEU_mps_f, targetSpeedNE_mps_f, clampAccuracy_mps_f, floatEpsilon_f);
    posVelSpNEU_mps_f = clamp_to_u_norm(posVelSpNEU_mps_f, maxAllowedSpeedU_mps_f, clampAccuracy_mps_f, floatEpsilon_f);

    if velNEValid_b
        rawVelSpNEU_mps_f(1:2) = rawVelSpNEU_mps_f(1:2) + posVelSpNEU_mps_f(1:2);
    else
        rawVelSpNEU_mps_f(1:2) = posVelSpNEU_mps_f(1:2);
    end

    if velUValid_b
        rawVelSpNEU_mps_f(3) = rawVelSpNEU_mps_f(3) + posVelSpNEU_mps_f(3);
    else
        rawVelSpNEU_mps_f(3) = posVelSpNEU_mps_f(3);
    end

elseif posNEValid_b
    %% 仅NE位置有效：生成二维水平位置速度目标
    waypointsNEU_m_f = [preWpNEU_m_f, curWpNEU_m_f, nextWpNEU_m_f];

    [crossingPointNEU_m_f, targetSpeedNE_mps_f, preMaxSpeedNEState_mps_f] = get_xy_guidance_constraints_handle(trajPosStateNEU_m_f, trajVelStateNEU_mps_f, waypointsNEU_m_f, ...
        isHoverWp_b, maxRouteSpeedNE_mps_f, maxJerkNE_mps3_f, maxAccNE_mps2_f, horizonAptRadius_m_f, minLookaheadDist_m_f, turnMinSpeed_mps_f, ...
        turnCosThreshold_f, turnJudgeDistState_m_f, turnPassSpeedState_mps_f, preMaxSpeedNEState_mps_f, smallValue_f);

    posToCrossingNE_m_f = crossingPointNEU_m_f(1:2) - trajPosStateNEU_m_f(1:2);
    directionToCrossingNE_f = unit_or_zero(posToCrossingNE_m_f, smallValue_f);
    posVelSpNE_mps_f = directionToCrossingNE_f * targetSpeedNE_mps_f;

    if velNEValid_b
        rawVelSpNEU_mps_f(1:2) = rawVelSpNEU_mps_f(1:2) + posVelSpNE_mps_f;
    else
        rawVelSpNEU_mps_f(1:2) = posVelSpNE_mps_f;
    end

elseif posUValid_b
    %% 仅U位置有效：生成一维垂向位置速度目标
    if isHoverWp_b
        nextWpForUSpeed_m_f = curWpNEU_m_f(3);
    else
        nextWpForUSpeed_m_f = nextWpNEU_m_f(3);
    end

    maxAllowedSpeedU_mps_f = get_max_z_speed_handle(trajPosStateNEU_m_f(3), curWpNEU_m_f(3), nextWpForUSpeed_m_f, maxJerkU_mps3_f, maxAccUp_mps2_f, maxAccDown_mps2_f, ...
        maxVelUp_mps_f, maxVelDown_mps_f, verticalAcceptanceRadius_m_f, smallValue_f);

    posErrorU_m_f = curWpNEU_m_f(3) - trajPosStateNEU_m_f(3);
    posVelSpU_mps_f = single(0.0);

    if abs(posErrorU_m_f) > smallValue_f
        posVelSpU_mps_f = sign(posErrorU_m_f) * maxAllowedSpeedU_mps_f;
    end

    if velUValid_b
        rawVelSpNEU_mps_f(3) = rawVelSpNEU_mps_f(3) + posVelSpU_mps_f;
    else
        rawVelSpNEU_mps_f(3) = posVelSpU_mps_f;
    end

else
    % 不处理，直接使用前馈速度
end

% 位置速度和速度前馈相加后，统一执行最终性能包线保护。
rawVelSpNEU_mps_f(1:2) = limit_vector_2d(rawVelSpNEU_mps_f(1:2), maxVelNE_mps_f, smallValue_f);     % 超长放缩
rawVelSpNEU_mps_f(3) = constrain_scalar(rawVelSpNEU_mps_f(3), -maxVelDown_mps_f, maxVelUp_mps_f);

%% 选择当前垂向整套约束
% NEU中U向上为正：rawVelSpU>0选择爬升约束，rawVelSpU<0选择下降约束。
if rawVelSpNEU_mps_f(3) > smallValue_f
    selectedUConstraintModeState_i8 = int8(1);
elseif rawVelSpNEU_mps_f(3) < -smallValue_f
    selectedUConstraintModeState_i8 = int8(-1);
else
    % 保持上一周期所选模式，使停车S曲线沿用进入停车前的整套参数。
end

if selectedUConstraintModeState_i8 > int8(0)
    selectedMaxAccU_mps2_f = maxAccUp_mps2_f;
    selectedMaxVelU_mps_f = maxVelUp_mps_f;
elseif selectedUConstraintModeState_i8 < int8(0)
    selectedMaxAccU_mps2_f = maxAccDown_mps2_f;
    selectedMaxVelU_mps_f = maxVelDown_mps_f;
else
    selectedMaxAccU_mps2_f = min(maxAccUp_mps2_f, maxAccDown_mps2_f);
    selectedMaxVelU_mps_f = min(maxVelUp_mps_f, maxVelDown_mps_f);
end

axisMaxAccPlanNEU_mps2_f = single([maxAccNE_mps2_f; maxAccNE_mps2_f; selectedMaxAccU_mps2_f]);
axisMaxVelPlanNEU_mps_f = single([maxVelNE_mps_f; maxVelNE_mps_f; selectedMaxVelU_mps_f]);

%% 计算三轴公共时间拉伸系数
% 水平：只有虚拟轨迹处于实际飞机运动前方时才进行时间拉伸。
timeStretchNE_f = single(1.0);
droneToTrajNE_m_f = trajPosStateNEU_m_f(1:2) - curPosNEU_m_f(1:2);
trajSpeedNE_mps_f = norm(trajVelStateNEU_mps_f(1:2));
trajectoryAheadNE_b = trajSpeedNE_mps_f > smallValue_f && dot(droneToTrajNE_m_f, trajVelStateNEU_mps_f(1:2)) > single(0.0);

if trajectoryAheadNE_b
    normalizedErrorNE_f = norm(droneToTrajNE_m_f) / maxTrajErrorNE_m_f;
    timeStretchNE_f = single(1.0) - constrain_scalar(normalizedErrorNE_f, single(0.0), single(1.0));
end

% 垂向：误差方向与轨迹速度方向一致，说明虚拟轨迹处于实际飞机前方。
timeStretchU_f = single(1.0);
droneToTrajU_m_f = trajPosStateNEU_m_f(3) - curPosNEU_m_f(3);
trajectoryAheadU_b = abs(trajVelStateNEU_mps_f(3)) > smallValue_f && droneToTrajU_m_f * trajVelStateNEU_mps_f(3) > single(0.0);

if trajectoryAheadU_b
    normalizedErrorU_f = abs(droneToTrajU_m_f) / maxTrajErrorU_m_f;
    timeStretchU_f = single(1.0) - constrain_scalar(normalizedErrorU_f, single(0.0), single(1.0));
end

% 三轴必须使用同一个有效时间推进，否则会破坏同步后的T1/T2/T3关系。
timeStretchNEU_f = min(timeStretchNE_f, timeStretchU_f);

%% 根据当前状态和本周期原始速度目标规划S曲线
trajVelSpNEU_mps_f = single(zeros(3,1));
trajDirectionNEU_f = single(zeros(3,1));
trajT1NEU_s_f = single(zeros(3,1));
trajT2NEU_s_f = single(zeros(3,1));
trajT3NEU_s_f = single(zeros(3,1));

for axisIdx_i = 1:3
    [trajVelSpNEU_mps_f(axisIdx_i), trajDirectionNEU_f(axisIdx_i), ...
        trajT1NEU_s_f(axisIdx_i), trajT2NEU_s_f(axisIdx_i), trajT3NEU_s_f(axisIdx_i)] = ...
        update_axis_durations(trajAccStateNEU_mps2_f(axisIdx_i), trajVelStateNEU_mps_f(axisIdx_i), rawVelSpNEU_mps_f(axisIdx_i), axisMaxVelPlanNEU_mps_f(axisIdx_i), ...
        axisMaxAccPlanNEU_mps2_f(axisIdx_i), axisMaxJerkNEU_mps3_f(axisIdx_i), smallValue_f);
end

%% N/E/U三轴时间同步
[trajT1NEU_s_f, trajT2NEU_s_f, trajT3NEU_s_f] = synchronize_trajectory_time_neu(trajT1NEU_s_f, trajT2NEU_s_f, trajT3NEU_s_f, trajAccStateNEU_mps2_f, trajVelStateNEU_mps_f, ...
trajVelSpNEU_mps_f, trajDirectionNEU_f, axisMaxAccPlanNEU_mps2_f, axisMaxJerkNEU_mps3_f, smallValue_f);

%% 用本周期刚得到的同步S曲线推进dt，并保存最小物理状态
trajJerkNEU_mps3_f = single(zeros(3,1));

for axisIdx_i = 1:3
    [trajJerkNEU_mps3_f(axisIdx_i), trajAccStateNEU_mps2_f(axisIdx_i), trajVelStateNEU_mps_f(axisIdx_i), trajPosStateNEU_m_f(axisIdx_i)] = ...
        update_trajectory_axis(trajAccStateNEU_mps2_f(axisIdx_i), trajVelStateNEU_mps_f(axisIdx_i), trajPosStateNEU_m_f(axisIdx_i), trajT1NEU_s_f(axisIdx_i), trajT2NEU_s_f(axisIdx_i), ...
        trajT3NEU_s_f(axisIdx_i), axisMaxJerkNEU_mps3_f(axisIdx_i), trajDirectionNEU_f(axisIdx_i), dtEff_s_f, timeStretchNEU_f);
end

%% 输出本周期推进后的轨迹状态
trajPosNEU_m_f = trajPosStateNEU_m_f;
trajVelNEU_mps_f = trajVelStateNEU_mps_f;
trajAccNEU_mps2_f = trajAccStateNEU_mps2_f;

end

function maxAllowedSpeedU_mps_f = get_max_z_speed_handle(trajPosU_m_f, curWpU_m_f, nextWpU_m_f, maxJerkU_mps3_f, maxAccUp_mps2_f, maxAccDown_mps2_f, ...
    maxVelUp_mps_f, maxVelDown_mps_f, verticalAcceptanceRadius_m_f, smallValue_f)
%#codegen
%
% 根据位置生成速度目标的方向，选择同方向轨迹所使用的整套加速度约束。
% 选中后，get_max_z_speed和后续S曲线均把该值作为对称加速度幅值。
% 不能因为爬升末段需要负加速度刹车，就切换为下降轨迹约束。

posErrorU_m_f = curWpU_m_f - trajPosU_m_f;

if posErrorU_m_f > smallValue_f
    maxAccSelectedU_mps2_f = maxAccUp_mps2_f;
elseif posErrorU_m_f < -smallValue_f
    maxAccSelectedU_mps2_f = maxAccDown_mps2_f;
else
    % 当前高度误差很小时，根据下一航段速度目标方向选择约束。
    nextSegmentDeltaU_m_f = nextWpU_m_f - curWpU_m_f;

    if nextSegmentDeltaU_m_f > smallValue_f
        maxAccSelectedU_mps2_f = maxAccUp_mps2_f;
    elseif nextSegmentDeltaU_m_f < -smallValue_f
        maxAccSelectedU_mps2_f = maxAccDown_mps2_f;
    else
        maxAccSelectedU_mps2_f = min(maxAccUp_mps2_f, maxAccDown_mps2_f);
    end
end

maxAllowedSpeedU_mps_f = get_max_z_speed(trajPosU_m_f, curWpU_m_f, nextWpU_m_f, maxJerkU_mps3_f, maxAccSelectedU_mps2_f, maxVelUp_mps_f, ...
    maxVelDown_mps_f, verticalAcceptanceRadius_m_f, smallValue_f);

end

function [crossingPointNEU_m_f, targetSpeedNE_mps_f, previousMaxSpeedNEOut_mps_f] = get_xy_guidance_constraints_handle(trajPosNEU_m_f, trajVelNEU_mps_f, waypointsNEU_m_f, ...
    isHoverWp_b, maxRouteSpeedNE_mps_f, maxJerkNE_mps3_f, maxAccNE_mps2_f, horizonAptRadius_m_f, minLookaheadDist_m_f, turnMinSpeed_mps_f, ...
    turnCosThreshold_f, turnJudgeDist_m_f, turnPassSpeed_mps_f, previousMaxSpeedNEIn_mps_f, smallValue_f)
%#codegen
%
% 统一生成3D和2D位置分支共用的水平追踪点及允许速度。
%
% 悬停航点：
%   以当前航点为目标，按剩余距离递推停车速度，最终速度为0。
%
% 快速航点：
%   maxRouteSpeedNE_mps_f只作为速度上限。
%   turnPassSpeed_mps_f为当前航点允许通过速度。
%   turnJudgeDist_m_f为mcLineJudge使用的提前分界面距离。
%   根据到分界面的剩余距离递推当前允许速度，使轨迹在进入转弯前
%   已经降低到turnPassSpeed_mps_f。

curWpNEU_m_f = waypointsNEU_m_f(:,2);

if isHoverWp_b
    crossingPointNEU_m_f = curWpNEU_m_f;

    distanceToTargetNE_m_f = norm(curWpNEU_m_f(1:2) - trajPosNEU_m_f(1:2));
    maxStopSpeedNE_mps_f = compute_max_speed_from_distance(maxJerkNE_mps3_f, maxAccNE_mps2_f, distanceToTargetNE_m_f, single(0.0), smallValue_f);
    targetSpeedNE_mps_f = min(maxRouteSpeedNE_mps_f, maxStopSpeedNE_mps_f);

else
    crossingPointNEU_m_f = get_crossing_point(trajPosNEU_m_f, trajVelNEU_mps_f, waypointsNEU_m_f, horizonAptRadius_m_f, minLookaheadDist_m_f, ...
        turnMinSpeed_mps_f, turnCosThreshold_f, smallValue_f);

    % 使用A->B方向计算虚拟轨迹点到提前分界面的沿程剩余距离。
    inVecNE_m_f = curWpNEU_m_f(1:2) - waypointsNEU_m_f(1:2,1);
    inLength_m_f = norm(inVecNE_m_f);

    if inLength_m_f > smallValue_f
        inDirNE_f = inVecNE_m_f / inLength_m_f;
        trajAlong_m_f = dot(trajPosNEU_m_f(1:2) - waypointsNEU_m_f(1:2,1), inDirNE_f);
        remainToWp_m_f = inLength_m_f - trajAlong_m_f;
        remainToTurnEntry_m_f = max(remainToWp_m_f - turnJudgeDist_m_f, single(0.0));

        maxSpeedByDistance_mps_f = compute_max_speed_from_distance(maxJerkNE_mps3_f, maxAccNE_mps2_f, remainToTurnEntry_m_f, turnPassSpeed_mps_f, smallValue_f);
        targetSpeedNE_mps_f = min(maxRouteSpeedNE_mps_f, maxSpeedByDistance_mps_f);
    else
        targetSpeedNE_mps_f = turnPassSpeed_mps_f;
    end
end

% 航段切换以后，当前pre-cur-next已经变为下一组航点。
% 此时新的速度递推可能允许重新加速，但飞机仍处于上一航点的转弯过程。
% 利用原有previousMaxSpeed状态，在转弯完成前禁止速度回升。
turning_b = is_turning(trajPosNEU_m_f, trajVelNEU_mps_f, curWpNEU_m_f, horizonAptRadius_m_f, turnMinSpeed_mps_f, turnCosThreshold_f, smallValue_f);

if ~isHoverWp_b && turning_b
    if previousMaxSpeedNEIn_mps_f > smallValue_f
        targetSpeedNE_mps_f = min(previousMaxSpeedNEIn_mps_f, targetSpeedNE_mps_f);
    end
end

previousMaxSpeedNEOut_mps_f = targetSpeedNE_mps_f;

end

function outputNEU_mps_f = clamp_to_xy_norm(inputNEU_mps_f, maxNormNE_mps_f, accuracy_mps_f, floatEpsilon_f)
%#codegen
%
% 1. 一般超限时按同一比例缩放整个NEU向量，保持三维方向不变；
% 2. 当水平上限和当前水平模长均小于accuracy时，只缩放NE分量，
%    避免微小水平数值误差把有效U速度一并缩小；

outputNEU_mps_f = inputNEU_mps_f;
normNEU_mps_f = norm(inputNEU_mps_f(1:2));
scaleFactor_f = single(1.0);

if normNEU_mps_f > floatEpsilon_f
    scaleFactor_f = maxNormNE_mps_f / normNEU_mps_f;
end

if scaleFactor_f < single(1.0)
    if maxNormNE_mps_f < accuracy_mps_f && normNEU_mps_f < accuracy_mps_f
        outputNEU_mps_f(1:2) = inputNEU_mps_f(1:2) * scaleFactor_f;
    else
        outputNEU_mps_f = inputNEU_mps_f * scaleFactor_f;
    end
end

end

function outputNEU_mps_f = clamp_to_u_norm(inputNEU_mps_f, maxNormU_mps_f, accuracy_mps_f, floatEpsilon_f)
%#codegen
%
% 1. 一般超限时按同一比例缩放整个NEU向量，保持三维方向不变；
% 2. 当垂向上限和当前垂向模长均小于accuracy时，只缩放U分量，
%    避免微小垂向数值误差把有效NE速度一并缩小。

outputNEU_mps_f = inputNEU_mps_f;
absSpeedU_mps_f = abs(inputNEU_mps_f(3));
scaleFactor_f = single(1.0);

if absSpeedU_mps_f > floatEpsilon_f
    scaleFactor_f = maxNormU_mps_f / absSpeedU_mps_f;
end

if scaleFactor_f < single(1.0)
    if maxNormU_mps_f < accuracy_mps_f && absSpeedU_mps_f < accuracy_mps_f
        outputNEU_mps_f(3) = inputNEU_mps_f(3) * scaleFactor_f;
    else
        outputNEU_mps_f = inputNEU_mps_f * scaleFactor_f;
    end
end

end

== matlab function GuidanceLaw/Subsystem/wpMssnHandle/GuiLaw/mcSpdGuidance/mcHorizonPosGuidance/horizonPosGuidance ==
  data: trajPosNE_m_f input; velCmdNE_mps_f output; trajVelNE_mps_f input; posNE_m_f input; kpPosNE_per_s_f input; maxVelNE_mps_f input
function velCmdNE_mps_f = horizonPosGuidance(trajPosNE_m_f, trajVelNE_mps_f, posNE_m_f, kpPosNE_per_s_f, maxVelNE_mps_f)
%#codegen
%
% 功能：
% 1. 根据虚拟轨迹位置与实际位置之差生成位置反馈速度；
% 2. 将虚拟轨迹速度作为速度前馈；
% 3. 水平合速度超限时优先保留位置反馈，剩余裕度分配给速度前馈。
%
% 输入：
%   trajPosNE_m_f      [2x1] 虚拟轨迹水平位置，m
%   trajVelNE_mps_f    [2x1] 虚拟轨迹水平速度前馈，m/s
%   posNE_m_f          [2x1] 飞行器实际水平位置，m
%   kpPosNE_per_s_f    [2x1] N、E方向位置反馈增益，1/s
%   maxVelNE_mps_f     [1x1] 最大允许水平合速度，m/s
%
% 输出：
%   velCmdNE_mps_f     [2x1] 水平速度指令，m/s

%% 位置反馈速度

positionErrorNE_m_f = trajPosNE_m_f - posNE_m_f;

positionFeedbackNE_mps_f = kpPosNE_per_s_f .* positionErrorNE_m_f;

%% 轨迹速度前馈与位置反馈合成

velCmdNE_mps_f = constrainNEPriority(positionFeedbackNE_mps_f, trajVelNE_mps_f, maxVelNE_mps_f);

end

function outputNE_mps_f = constrainNEPriority(posFeedbackNE_mps_f, velFeedforwardNE_mps_f, maxVelNE_mps_f)
%#codegen
%
% 优先级：
%   位置反馈速度 > 轨迹速度前馈。
%
% 限幅原则：
% 1. 两者之和未超限时全部保留；
% 2. 位置反馈本身超限时，只保留限幅后的位置反馈；
% 3. 其余情况下完整保留位置反馈，仅缩小轨迹速度前馈幅值。

smallValue_f = single(1.0e-3);

% outputNE_mps_f = single(zeros(2, 1));

%% 两部分速度均可完整保留

combinedNE_mps_f = posFeedbackNE_mps_f + velFeedforwardNE_mps_f;

if norm(combinedNE_mps_f) <= maxVelNE_mps_f
    outputNE_mps_f = combinedNE_mps_f;
    return;
end

%% 位置反馈本身已经达到水平速度限制

posFeedbackNorm_mps_f = norm(posFeedbackNE_mps_f);

if posFeedbackNorm_mps_f >= maxVelNE_mps_f
    outputNE_mps_f = posFeedbackNE_mps_f * (maxVelNE_mps_f / posFeedbackNorm_mps_f);
    return;
end


%% 轨迹速度前馈接近零

velFeedforwardNorm_mps_f = norm(velFeedforwardNE_mps_f);

if velFeedforwardNorm_mps_f <= smallValue_f
    outputNE_mps_f = posFeedbackNE_mps_f;
    return;
end

%% 完整保留位置反馈，并计算轨迹速度前馈的允许幅值

velFeedforwardNE_unit_f = velFeedforwardNE_mps_f / velFeedforwardNorm_mps_f;

parallelSpeed_mps_f = dot(velFeedforwardNE_unit_f, posFeedbackNE_mps_f);

constantTerm_mps2_f = dot(posFeedbackNE_mps_f, posFeedbackNE_mps_f) - maxVelNE_mps_f * maxVelNE_mps_f;

radicand_mps2_f = parallelSpeed_mps_f * parallelSpeed_mps_f - constantTerm_mps2_f;
radicand_mps2_f = max(radicand_mps2_f, single(0.0));

allowedFeedforwardSpeed_mps_f = -parallelSpeed_mps_f + sqrt(radicand_mps2_f);

allowedFeedforwardSpeed_mps_f = min(max(allowedFeedforwardSpeed_mps_f, single(0.0)), velFeedforwardNorm_mps_f);

outputNE_mps_f = posFeedbackNE_mps_f + allowedFeedforwardSpeed_mps_f * velFeedforwardNE_unit_f;

%% 消除单精度舍入可能造成的极小速度越界

outputNorm_mps_f = norm(outputNE_mps_f);

if outputNorm_mps_f > maxVelNE_mps_f
    outputNE_mps_f = outputNE_mps_f * (maxVelNE_mps_f / outputNorm_mps_f);
end

end

== matlab function GuidanceLaw/Subsystem/wpMssnHandle/GuiLaw/fwVertSpdGuidance/fwVertSpdGuidance ==
  data: curPosNEU_m_f input; vuCmd_mps_f output; velNEU_mps_f input; wpPreNEU_m_f input; curWp_struct input; segSwitch_b input; dt_s_f input; reset_b input; param_f input
function vuCmd_mps_f = fwVertSpdGuidance(curPosNEU_m_f, velNEU_mps_f, wpPreNEU_m_f, curWp_struct, segSwitch_b, dt_s_f, reset_b, param_f)
%#codegen
%
% 固定翼垂向速度指令生成导引算法
%
% param_f：
% 1  最大爬升率，m/s
% 2  最大下降率绝对值，m/s
% 3  高度误差反馈增益，1/s
% 4  垂速向上变化率，m/s^2
% 5  垂速向下变化率，m/s^2
% 6  航点提前切换距离，m
% 7  最小有效水平航段长度，m

persistent vertSpdCmdState_mps_f
persistent pathProgressState_f

firstRun_b = false;

if isempty(vertSpdCmdState_mps_f)
    vertSpdCmdState_mps_f = single(0.0);
    firstRun_b = true;
end

if isempty(pathProgressState_f)
    pathProgressState_f = single(0.0);
    firstRun_b = true;
end

%% 参数解析
smallValue_f = single(1.0e-6);

climbRateMax_mps_f = max(abs(param_f(1)), single(0.0));
sinkRateMax_mps_f = max(abs(param_f(2)), single(0.0));
altitudeGain_f = max(param_f(3), single(0.0));
vertAccUpMax_mps2_f = max(abs(param_f(4)), single(0.0));
vertAccDownMax_mps2_f = max(abs(param_f(5)), single(0.0));
switchLeadDist_m_f = max(param_f(6), single(0.0));
minHorizontalLength_m_f = max(param_f(7), smallValue_f);

dtUse_s_f = max(dt_s_f, single(0.0));

resetState_b = reset_b || firstRun_b;

vuMin_mps_f = -sinkRateMax_mps_f;
vuMax_mps_f = climbRateMax_mps_f;

%% 当前目标航点
wpTargetNEU_m_f = [curWp_struct.posN_m_f; curWp_struct.posE_m_f; curWp_struct.posU_m_f];

%% 判断是否为直线航段，5:圆弧航段
if curWp_struct.wpType_u8 == uint8(5)
    isStraight_b = false;
else
    isStraight_b = true;
end

%% 初始化直线航段计算变量

segmentNE_m_f = [single(0.0); single(0.0)];
segmentLength_m_f = single(0.0);
effectivePathLength_m_f = single(0.0);
useLinePath_b = false;

if isStraight_b == true
    segmentNE_m_f = wpTargetNEU_m_f(1:2) - wpPreNEU_m_f(1:2);
    segmentLength_m_f = norm(segmentNE_m_f);
    effectivePathLength_m_f = max(segmentLength_m_f - switchLeadDist_m_f, single(0.0));
    if effectivePathLength_m_f > minHorizontalLength_m_f
        useLinePath_b = true;
    else
        useLinePath_b = false;
    end
    
end

%% 1. 生成垂速目标
if useLinePath_b
    %% 1.1 直线航段路径高度跟踪
    tangentNE_f = segmentNE_m_f / segmentLength_m_f;

    fromPrevNE_m_f = curPosNEU_m_f(1:2) - wpPreNEU_m_f(1:2);
    alongTrack_m_f = dot(fromPrevNE_m_f, tangentNE_f);

    pathProgressMeasured_f = constrain_scalar(alongTrack_m_f / effectivePathLength_m_f, single(0.0), single(1.0));

    if resetState_b || segSwitch_b
        % 航段切换时，以当前位置投影进度初始化
        pathProgressState_f = pathProgressMeasured_f;
    else
        % 防止飞机短时后退导致高度参考反向移动
        pathProgressState_f = max(pathProgressState_f, pathProgressMeasured_f);
    end

    groundSpeedAlong_mps_f = dot(velNEU_mps_f(1:2), tangentNE_f);
    groundSpeedAlong_mps_f = max(groundSpeedAlong_mps_f, single(0.0));

    pathProgressRate_f = groundSpeedAlong_mps_f / effectivePathLength_m_f;

    if alongTrack_m_f < single(0.0) || pathProgressState_f >= single(1.0)
        pathProgressRate_f = single(0.0);
    end

    altitudeDelta_m_f = wpTargetNEU_m_f(3) - wpPreNEU_m_f(3);
    pathAltitude_m_f = wpPreNEU_m_f(3) + altitudeDelta_m_f * pathProgressState_f;

    vertSpdFeedforward_mps_f = altitudeDelta_m_f * pathProgressRate_f;
    vertSpdFeedback_mps_f = altitudeGain_f * (pathAltitude_m_f - curPosNEU_m_f(3));

    vertSpdTarget_mps_f = vertSpdFeedforward_mps_f + vertSpdFeedback_mps_f;

else
    %% 1.2 圆弧航段或水平航段过短
    altitudeError_m_f = wpTargetNEU_m_f(3) - curPosNEU_m_f(3);

    vertSpdTarget_mps_f = altitudeCaptureSpeed(altitudeError_m_f, altitudeGain_f, climbRateMax_mps_f, sinkRateMax_mps_f, vertAccUpMax_mps2_f, vertAccDownMax_mps2_f, smallValue_f);

    pathProgressState_f = single(0.0);
end

%% 2. 垂速包线限制
vertSpdRaw_mps_f = constrain_scalar(vertSpdTarget_mps_f, vuMin_mps_f, vuMax_mps_f);

%% 3. 垂速变化率限制
if resetState_b
    % 初始化为当前实际垂速，避免使能瞬间发生跳变
    vertSpdCmdState_mps_f = constrain_scalar(velNEU_mps_f(3), vuMin_mps_f, vuMax_mps_f);
else
    vertSpdCmdState_mps_f = rateLimit(vertSpdRaw_mps_f, vertSpdCmdState_mps_f, vertAccUpMax_mps2_f, vertAccDownMax_mps2_f, dtUse_s_f);
    vertSpdCmdState_mps_f = constrain_scalar(vertSpdCmdState_mps_f, vuMin_mps_f, vuMax_mps_f);
end

vuCmd_mps_f = vertSpdCmdState_mps_f;

end

%% ------------------------------------------------------------------------
function vertSpdTarget_mps_f = altitudeCaptureSpeed(altitudeError_m_f, altitudeGain_f, climbRateMax_mps_f, sinkRateMax_mps_f, vertAccUpMax_mps2_f, vertAccDownMax_mps2_f, smallValue_f)
%#codegen
%
% 根据高度误差生成带制动距离约束的垂速目标

if altitudeError_m_f > single(0.0)
    %% 爬升
    vertSpdByGain_mps_f = altitudeGain_f * altitudeError_m_f;

    % 正爬升速度减小到零时，使用向下变化率计算制动速度
    brakeAcc_mps2_f = max(vertAccDownMax_mps2_f, smallValue_f);
    vertSpdByBrake_mps_f = sqrt(single(2.0) * brakeAcc_mps2_f * altitudeError_m_f);

    vertSpdTarget_mps_f = min(vertSpdByGain_mps_f, vertSpdByBrake_mps_f);
    vertSpdTarget_mps_f = min(vertSpdTarget_mps_f, climbRateMax_mps_f);

elseif altitudeError_m_f < single(0.0)
    %% 下降
    altitudeErrorAbs_m_f = abs(altitudeError_m_f);
    sinkSpdByGain_mps_f = altitudeGain_f * altitudeErrorAbs_m_f;

    % 负下降速度恢复到零时，使用向上变化率计算制动速度
    brakeAcc_mps2_f = max(vertAccUpMax_mps2_f, smallValue_f);
    sinkSpdByBrake_mps_f = sqrt(single(2.0) * brakeAcc_mps2_f * altitudeErrorAbs_m_f);

    sinkRateTarget_mps_f = min(sinkSpdByGain_mps_f, sinkSpdByBrake_mps_f);
    sinkRateTarget_mps_f = min(sinkRateTarget_mps_f, sinkRateMax_mps_f);

    vertSpdTarget_mps_f = -sinkRateTarget_mps_f;

else
    vertSpdTarget_mps_f = single(0.0);
end

end
